simulink model "PMSMBridgeBusPlant"  (R2026b)
settings: Solver=VariableStepAuto
undefined symbols (not defined in the file or in its folder): pmsm_bridge_parameters
settings Model: Creator=24322  LastModifiedBy=24322

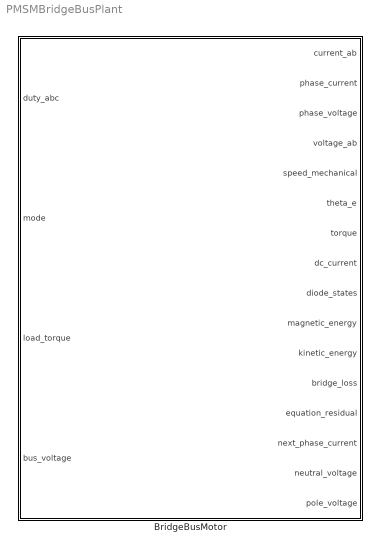
== system PMSMBridgeBusPlant ==
  BridgeBusMotor : Subsystem  mask{cfg=pmsm_bridge_parameters()}
      mask prompts: cfg "Physical bridge/PMSM configuration"

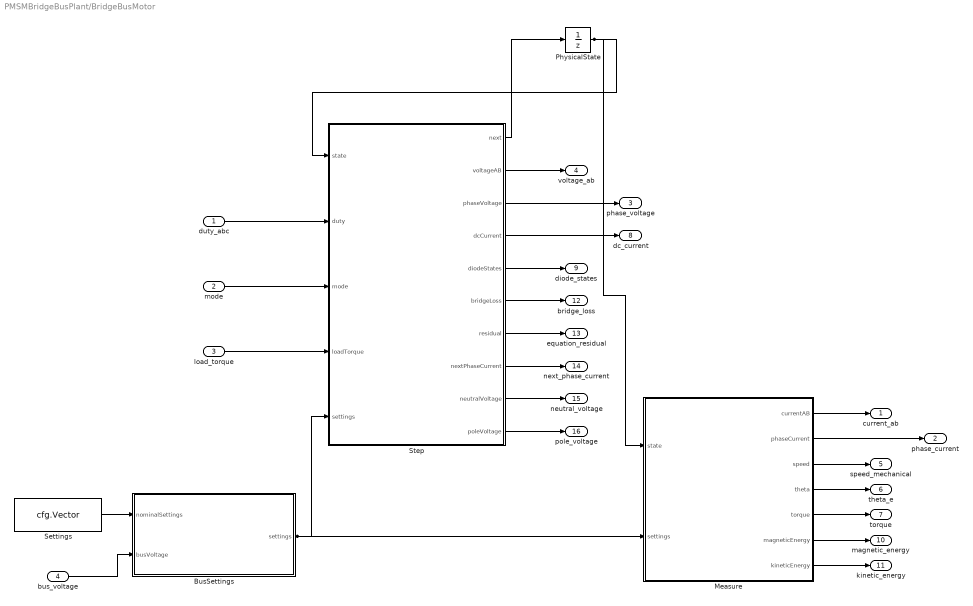
== system PMSMBridgeBusPlant/BridgeBusMotor ==
  duty_abc : Inport  SampleTime=cfg.Ts
  mode : Inport  Port=2  SampleTime=cfg.Ts
  load_torque : Inport  Port=3  SampleTime=cfg.Ts
  bus_voltage : Inport  Port=4  SampleTime=cfg.Ts
  BusSettings : MATLAB Function  TreatAsAtomicUnit=on
  Measure : MATLAB Function  TreatAsAtomicUnit=on
  PhysicalState : UnitDelay  InitialCondition=cfg.State0  SampleTime=cfg.Ts
  Settings : Constant  Value=cfg.Vector
  Step : MATLAB Function  TreatAsAtomicUnit=on
  current_ab : Outport
  phase_current : Outport  Port=2
  phase_voltage : Outport  Port=3
  voltage_ab : Outport  Port=4
  speed_mechanical : Outport  Port=5
  theta_e : Outport  Port=6
  torque : Outport  Port=7
  dc_current : Outport  Port=8
  diode_states : Outport  Port=9
  magnetic_energy : Outport  Port=10
  kinetic_energy : Outport  Port=11
  bridge_loss : Outport  Port=12
  equation_residual : Outport  Port=13
  next_phase_current : Outport  Port=14
  neutral_voltage : Outport  Port=15
  pole_voltage : Outport  Port=16
  wires:
  Step/10(poleVoltage) -> pole_voltage/1
  Step/9(neutralVoltage) -> neutral_voltage/1
  Step/8(nextPhaseCurrent) -> next_phase_current/1
  Step/7(residual) -> equation_residual/1
  Step/6(bridgeLoss) -> bridge_loss/1
  Step/5(diodeStates) -> diode_states/1
  Step/4(dcCurrent) -> dc_current/1
  Step/2(voltageAB) -> voltage_ab/1
  Step/3(phaseVoltage) -> phase_voltage/1
  Measure/7(kineticEnergy) -> kinetic_energy/1
  Measure/6(magneticEnergy) -> magnetic_energy/1
  Measure/5(torque) -> torque/1
  Measure/4(theta) -> theta_e/1
  Measure/3(speed) -> speed_mechanical/1
  Measure/2(phaseCurrent) -> phase_current/1
  Measure/1(currentAB) -> current_ab/1
  load_torque/1 -> Step/4(loadTorque)
  mode/1 -> Step/3(mode)
  duty_abc/1 -> Step/2(duty)
  Step/1(next) -> PhysicalState/1
  Settings/1 -> BusSettings/1(nominalSettings)
  PhysicalState/1 -> Measure/1(state), Step/1(state)
  bus_voltage/1 -> BusSettings/2(busVoltage)
  BusSettings/1(settings) -> Measure/2(settings), Step/5(settings)

== matlab function PMSMBridgeBusPlant/BridgeBusMotor/Measure ==
  data: state input; currentAB output; settings input; phaseCurrent output; speed output; theta output; torque output; magneticEnergy output; kineticEnergy output
function [currentAB,phaseCurrent,speed,theta,torque,magneticEnergy,kineticEnergy]=pmsm_bridge_output(state,settings)
%PMSM_BRIDGE_OUTPUT State-only physical outputs at the beginning of a step.
% state=[i_alpha;i_beta;omega_mechanical;theta_mechanical]. SI peak convention.
%#codegen
currentAB=state(1:2);speed=state(3);
angle=settings(6)*state(4);cosine=cos(angle);sine=sin(angle);
theta=atan2(sine,cosine);
id=cosine*currentAB(1)+sine*currentAB(2);
iq=-sine*currentAB(1)+cosine*currentAB(2);
torque=1.5*settings(6)*(settings(5)*iq+(settings(3)-settings(4))*id*iq);
phaseCurrent=[currentAB(1);-0.5*currentAB(1)+sqrt(3)/2*currentAB(2); ...
    -0.5*currentAB(1)-sqrt(3)/2*currentAB(2)];
magneticEnergy=0.75*(settings(3)*id*id+settings(4)*iq*iq);
kineticEnergy=0.5*settings(7)*speed*speed;
end

== matlab function PMSMBridgeBusPlant/BridgeBusMotor/Step ==
  data: state input; next output; duty input; mode input; loadTorque input; settings input; voltageAB output; phaseVoltage output; dcCurrent output; diodeStates output; bridgeLoss output; residual output; nextPhaseCurrent output; neutralVoltage output; poleVoltage output
function [next,voltageAB,phaseVoltage,dcCurrent,diodeStates,bridgeLoss,residual,nextPhaseCurrent,neutralVoltage,poleVoltage]=pmsm_bridge_step(state,duty,mode,loadTorque,settings)
%PMSM_BRIDGE_STEP Coupled linear PMSM + ideal PWM/PWL freewheel diode bridge.
% Mode: 0 all gates OFF (diode rectifier), 1 averaged PWM, 2 active short.
% Electrical flux balance uses backward Euler; mechanics uses forward Euler.
% Current outputs belong to state[k]. Solver voltages/current diagnostics
% describe the k -> k+1 interval; no current reset is used when gates turn off.
% settings=[Ts;Rs;Ld;Lq;Flux;p;J;B;Vdc;Vf;Ron;MechanicalEnabled; ...
%           CurrentTolerance;VoltageTolerance;MaxCurrent;MaxSpeed;MaxAngleStep].
%#codegen
assert(all(isfinite(state)) && all(isfinite(settings)) && isfinite(loadTorque));
assert(mode==0 || mode==1 || mode==2,'Bridge mode must be 0, 1 or 2.');
step=settings(1);rs=settings(2);ld=settings(3);lq=settings(4);
flux=settings(5);pairs=settings(6);inertia=settings(7);friction=settings(8);
bus=settings(9);vf=settings(10);ron=settings(11);
assert(step>0 && ld>0 && lq>0 && inertia>0 && bus>0 && rs>=0 && vf>=0 && ron>=0);
assert(max(abs(state(1:2)))<=settings(15) && abs(state(3))<=settings(16));
assert(abs(pairs*state(3)*step)<=settings(17),'Electrical angle increment exceeds configured model limit.');
angle=pairs*state(4);cosine=cos(angle);sine=sin(angle);
rotation=[cosine,-sine;sine,cosine];inductance=rotation*diag([ld,lq])*rotation';
magnet=flux*[cosine;sine];oldFlux=inductance*state(1:2)+magnet;
id=cosine*state(1)+sine*state(2);iq=-sine*state(1)+cosine*state(2);
torque=1.5*pairs*(flux*iq+(ld-lq)*id*iq);
next=zeros(4,1,'like',state);next(3)=state(3);
if settings(12)>0.5
    next(3)=state(3)+step*(torque-loadTorque-friction*state(3))/inertia;
end
next(4)=state(4)+step*state(3); % prescribed-speed mode also advances angle
futureAngle=pairs*next(4);futureCosine=cos(futureAngle);futureSine=sin(futureAngle);
futureRotation=[futureCosine,-futureSine;futureSine,futureCosine];
matrix=futureRotation*diag([ld,lq])*futureRotation'+step*rs*eye(2);
forcing=oldFlux-flux*[futureCosine;futureSine];
transform=[1,0;-0.5,sqrt(3)/2;-0.5,-sqrt(3)/2];
diodeStates=zeros(3,1,'like',state);neutralVoltage=zeros(1,'like',state);
if mode==0
    [current,voltageAB,poleVoltage,neutralVoltage,diodeStates]= ...
        solveRectifier(matrix,forcing,step,bus,vf,ron,settings(13),settings(14));
elseif mode==1
    assert(all(isfinite(duty)) && all(duty>=0) && all(duty<=1),'PWM duty must be finite in [0,1].');
    poleVoltage=bus*duty;neutralVoltage=sum(poleVoltage)/3;
    voltageAB=[(2*poleVoltage(1)-poleVoltage(2)-poleVoltage(3))/3; ...
        (poleVoltage(2)-poleVoltage(3))/sqrt(3)];
    current=matrix\(forcing+step*voltageAB);
else
    poleVoltage=zeros(3,1,'like',state);voltageAB=zeros(2,1,'like',state);
    current=matrix\forcing;
end
next(1:2)=current;nextPhaseCurrent=transform*current;phaseVoltage=transform*voltageAB;
dcCurrent=zeros(1,'like',state);bridgeLoss=zeros(1,'like',state);
if mode==1
    dcCurrent=sum(duty.*nextPhaseCurrent);
elseif mode==0
    for phaseIndex=1:3
        if diodeStates(phaseIndex)<-0.5,dcCurrent=dcCurrent+nextPhaseCurrent(phaseIndex);end
        if abs(diodeStates(phaseIndex))>0.5
            bridgeLoss=bridgeLoss+vf*abs(nextPhaseCurrent(phaseIndex))+ron*nextPhaseCurrent(phaseIndex)^2;
        end
    end
end
residual=max(abs((matrix*current-forcing)/step-voltageAB));
assert(all(isfinite(next)) && all(isfinite(voltageAB)) && all(isfinite(poleVoltage)));
assert(max(abs(next(1:2)))<=settings(15) && abs(next(3))<=settings(16),'Physical model range exceeded.');
end

function [current,voltage,poles,neutral,states]=solveRectifier(matrix,forcing,step,bus,vf,ron,currentTolerance,voltageTolerance)
% Current into a motor phase is positive. Lower diode: +1; upper: -1.
% Open phase current is zero and its pole voltage lies between -Vf and Vdc+Vf.
transform=[1,0;-0.5,sqrt(3)/2;-0.5,-sqrt(3)/2];
current=zeros(2,1,'like',forcing);states=zeros(3,1,'like',forcing);
voltage=-forcing/step;freePoles=transform*voltage;
low=-vf-min(freePoles);high=bus+vf-max(freePoles);
neutral=(low+high)/2;poles=freePoles+neutral;
if high>=low-voltageTolerance,return;end
% A balanced three-wire current has both signs. These twelve conducting
% patterns plus the all-open case cover every feasible diode configuration.
patterns=[1,-1,0;1,0,-1;-1,1,0;0,1,-1;-1,0,1;0,-1,1; ...
    1,1,-1;1,-1,1;-1,1,1;1,-1,-1;-1,1,-1;-1,-1,1];
impedance=matrix/step+ron*eye(2);source=forcing/step;found=false;
for patternIndex=1:12
    candidateStates=patterns(patternIndex,:)';system=zeros(3,3,'like',forcing);rhs=zeros(3,1,'like',forcing);
    for phaseIndex=1:3
        if candidateStates(phaseIndex)==0
            system(phaseIndex,1:2)=transform(phaseIndex,:);
        else
            system(phaseIndex,1:2)=transform(phaseIndex,:)*impedance;
            system(phaseIndex,3)=1;
            rail=-vf;if candidateStates(phaseIndex)<0,rail=bus+vf;end
            rhs(phaseIndex)=rail+transform(phaseIndex,:)*source;
        end
    end
    solution=system\rhs;candidate=solution(1:2);candidateNeutral=solution(3);
    candidateVoltage=(matrix*candidate-forcing)/step;
    candidatePoles=transform*candidateVoltage+candidateNeutral;phaseCurrent=transform*candidate;
    valid=true;
    for phaseIndex=1:3
        if candidateStates(phaseIndex)>0
            valid=valid && phaseCurrent(phaseIndex)>=-currentTolerance;
        elseif candidateStates(phaseIndex)<0
            valid=valid && phaseCurrent(phaseIndex)<=currentTolerance;
        else
            valid=valid && abs(phaseCurrent(phaseIndex))<=currentTolerance && ...
                candidatePoles(phaseIndex)>=-vf-voltageTolerance && candidatePoles(phaseIndex)<=bus+vf+voltageTolerance;
        end
    end
    if valid
        current=candidate;voltage=candidateVoltage;poles=candidatePoles;
        neutral=candidateNeutral;states=candidateStates;found=true;break
    end
end
assert(found,'No consistent diode conduction state.');
end

== matlab function PMSMBridgeBusPlant/BridgeBusMotor/BusSettings ==
  data: nominalSettings input; settings output; busVoltage input
function settings=bridge_bus_settings(nominalSettings,busVoltage)
%#codegen
%BRIDGE_BUS_SETTINGS Apply the measured/specified DC rail for this interval.
assert(isfinite(busVoltage) && busVoltage>0, ...
    'Positive finite DC bus voltage required.');
settings=nominalSettings;
settings(9)=busVoltage;
end
